simulink model "p_global_simulink_test_block"  (R2017a)
settings: Solver=ode45  StartTime=0.0  StopTime=0.1  RelTol=1e-3
settings Model: Creator=oj  LastModifiedBy=sandmann
settings DataIOCC: SaveFormat=StructureWithTime  ReturnWorkspaceOutputs=on
settings OptimizationCC: LifeSpan=inf
settings DebuggingCC: FcnCallInpInsideContextMsg=warning  SFExecutionAtInitializationDiag=none
settings HardwareCC: ProdBitPerSizeT=32  ProdBitPerPtrDiffT=32  ProdWordSize=32  ProdHWDeviceType=Specified
settings ModelReferenceCC: EnableRefExpFcnMdlSchedulingChecks=off
settings SFSimCC: SimUseLocalCustomCode=on
settings RTWCC: RTWUseLocalCustomCode=on

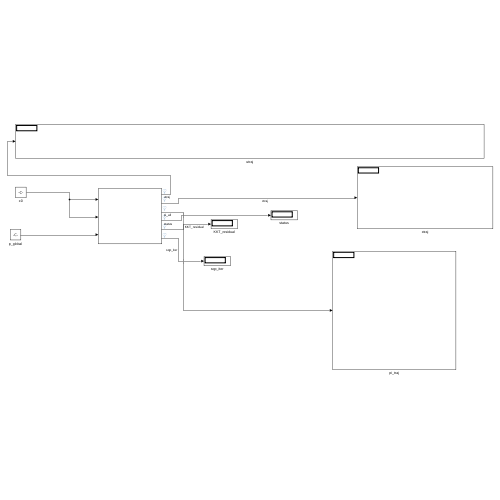
[thumbnail: Simulink's stored preview of the top-level diagram]
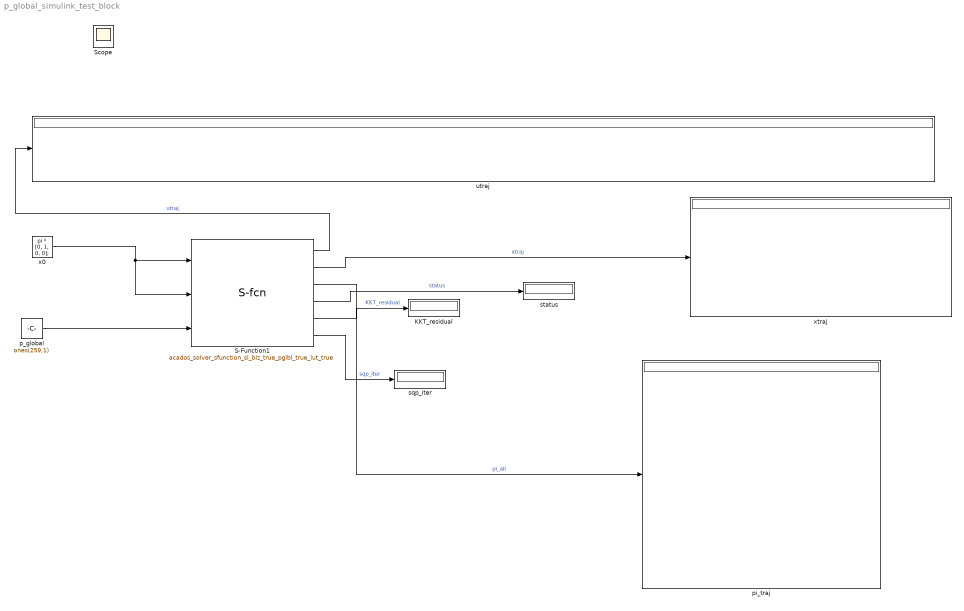
== system p_global_simulink_test_block ==
  KKT_residual : Display
  S-Function1 : S-Function  FunctionName=acados_solver_sfunction_sl_blz_true_pglbl_true_lut_true  SFunctionDeploymentMode=off  EnableBusSupport=off
      mask Display:
      | global sfun_input_names sfun_output_names
      | for i = 1:length(sfun_input_names)
      | 	port_label('input', i, sfun_input_names{i})
      | end
      | for i = 1:length(sfun_output_names)
      | 	port_label('output', i, sfun_output_names{i})
      | end
  p_global : Constant  Value=ones(259,1)
  pi_traj : Display
  sqp_iter : Display
  status : Display
  utraj : Display
  x0 : Constant  Value=pi * [0, 1, 0, 0];
  xtraj : Display
  Scope : Scope
  wires:
  S-Function1/5 -> KKT_residual/1  "KKT_residual"
  S-Function1/1 -> utraj/1  "utraj"
  x0/1 -> S-Function1/2, S-Function1/1
  S-Function1/2 -> xtraj/1  "xtraj"
  S-Function1/6 -> sqp_iter/1  "sqp_iter"
  S-Function1/4 -> status/1  "status"
  S-Function1/3 -> pi_traj/1  "pi_all"
  p_global/1 -> S-Function1/3
